simulink model "v0_pmsm_fsfb_sim_for_flipsky"  (R2025b)
settings: Solver=FixedStepAuto  StartTime=0.0  StopTime=inf  FixedStep=Ts_pwm  RelTol=1e-3
values from neighbouring files (symbols this model uses):
  Bv = pmsm.B    [mcb_pmsm_foc_qep_f28379d_SIUnit_data.m]    (also in mcb_pmsm_fsfb_f28379d_param.m = 2.636e-06; v0_pmsm_fsfb_sim_for_flipsky_.m = 9.444e-05; v1_0_3_sim_param_fsfc.m = 9.444e-05)
  C = [ 1, 0, 0 ... (first row only)    [mcb_pmsm_fsfb_f28379d_param.m]    (also in v0_pmsm_fsfb_sim_for_flipsky_.m = [; v1_0_3_sim_param_fsfc.m = [)
  J = 7.061e-6    (= 7.061e-06)    [mcb_pmsm_fsfb_f28379d_param.m]    (also in v0_pmsm_fsfb_sim_for_flipsky_.m = 0.00036179; v1_0_3_sim_param_fsfc.m = 0.00036179)
  Ki = -Ka_fsfb(2)    [mcb_pmsm_foc_qep_f28379d_SIUnit_data.m]    (also in mcb_pmsm_fsfb_f28379d_param.m = -K(:, n+1:end); v0_pmsm_fsfb_sim_for_flipsky_.m = -K(:, n+1:end); v1_0_3_sim_param_fsfc.m = -K(:, n+1:end))
  Kx = K(:, 1:n)    [mcb_pmsm_fsfb_f28379d_param.m]    (also in v0_pmsm_fsfb_sim_for_flipsky_.m; v1_0_3_sim_param_fsfc.m)
  L = Ld    (= 0.0002)    [mcb_pmsm_fsfb_f28379d_param.m]    (also in v0_pmsm_fsfb_sim_for_flipsky_.m = 0.0004; v1_0_3_sim_param_fsfc.m = 0.0013)
  Lambda_m = 0.01273    [mcb_pmsm_fsfb_f28379d_param.m]    (also in v0_pmsm_fsfb_sim_for_flipsky_.m = 0.0426; v1_0_3_sim_param_fsfc.m = 0.08627)
  P = 8    [mcb_pmsm_fsfb_f28379d_param.m]    (also in v0_pmsm_fsfb_sim_for_flipsky_.m; v1_0_3_sim_param_fsfc.m)
  Pk0 = 5e-4*diag([1e-3, 1e-2, 0.2, 0.01])    [v0_pmsm_fsfb_sim_for_flipsky_.m]    (also in v1_0_3_sim_param_fsfc.m)
  Qd = 1e-4*diag([0.5, 0.5, 5, 0.5])    [v0_pmsm_fsfb_sim_for_flipsky_.m]    (also in v1_0_3_sim_param_fsfc.m)
  R = Rs    (= 0.72)    [v0_pmsm_fsfb_sim_for_flipsky_.m]    (also in v1_0_3_sim_param_fsfc.m = 0.52)
  Rc = 56.33    [v0_pmsm_fsfb_sim_for_flipsky_.m]    (also in v1_0_3_sim_param_fsfc.m = 450)
  Rs = 0.3819    [mcb_pmsm_fsfb_f28379d_param.m]    (also in v0_pmsm_fsfb_sim_for_flipsky_.m = 0.72; v1_0_3_sim_param_fsfc.m = 0.52)
  Tc = 0.001    [v0_pmsm_fsfb_sim_for_flipsky_.m]    (also in v1_0_3_sim_param_fsfc.m)
  Ts = T_pwm    (= 5e-05)    [mcb_pmsm_foc_qep_f28379d_SIUnit_data.m]    (also in v0_pmsm_fsfb_sim_for_flipsky_.m = 0.0001; v1_0_3_sim_param_fsfc.m = 0.0001)
  X04 = 1e-2*[1; 1; 1; 0]    [v0_pmsm_fsfb_sim_for_flipsky_.m]    (also in v1_0_3_sim_param_fsfc.m)
libraries: simulink x4
settings Model: Creator=rotanakchhean  LastModifiedBy=LabPC

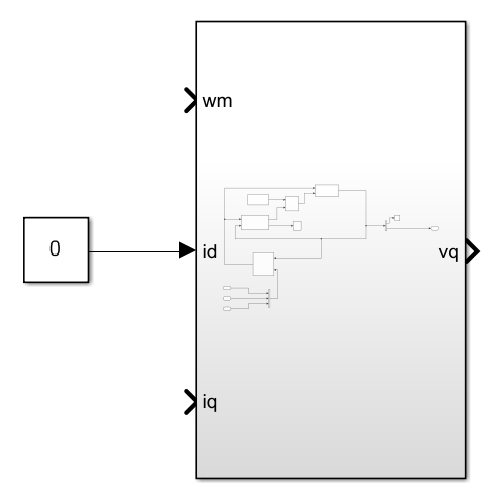
[thumbnail: Simulink's stored preview of the top-level diagram]
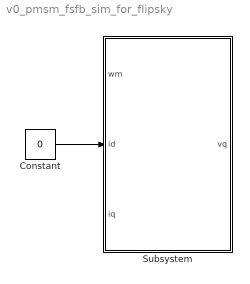
== system v0_pmsm_fsfb_sim_for_flipsky ==
  Constant : Constant  Value=0
  Subsystem : Subsystem
  wires:
  Constant/1 -> Subsystem/2(id)

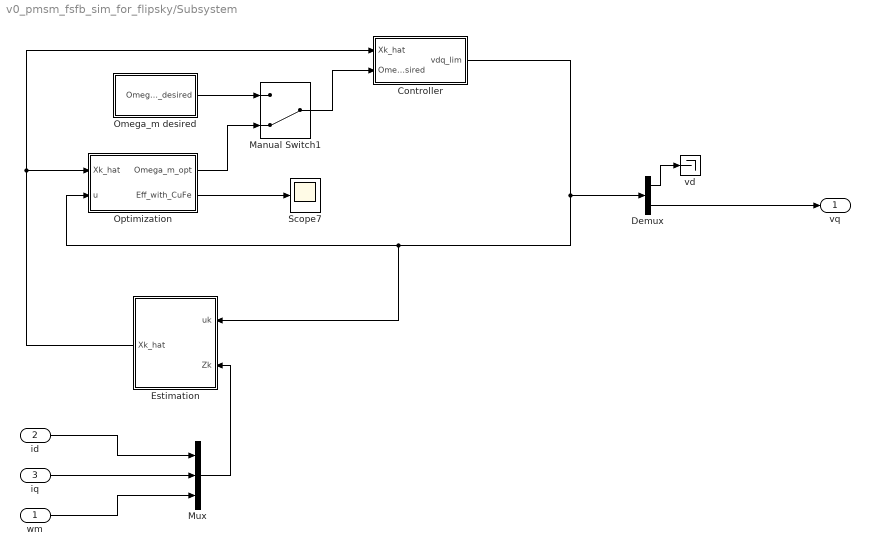
== system v0_pmsm_fsfb_sim_for_flipsky/Subsystem ==
  wm : Inport
  id : Inport  Port=2
  iq : Inport  Port=3
  Controller : Subsystem
  Demux : Demux  Outputs=2
  Estimation : Subsystem
  Manual Switch1 : ManualSwitch  CurrentSetting=0
  Mux : Mux  Inputs=3
  Omega_m desired : Subsystem
  Optimization : Subsystem
  Scope7 : Scope
      settings: ActiveDisplayYMinimum=-1.01629  ActiveDisplayYMaximum=1.19485
  vd : Terminator
  vq : Outport
  wires:
  Demux/2 -> vq/1
  wm/1 -> Mux/3
  Demux/1 -> vd/1
  Manual Switch1/1 -> Controller/2(Omega_m_desired)
  id/1 -> Mux/1
  Controller/1(vdq_lim) -> Demux/1, Optimization/2(u), Estimation/1(uk)
  Optimization/2(Eff_with_CuFe) -> Scope7/1
  Estimation/1(Xk_hat) -> Optimization/1(Xk_hat), Controller/1(Xk_hat)
  Optimization/1(Omega_m_opt) -> Manual Switch1/2
  Omega_m desired/1(Omega_m_desired) -> Manual Switch1/1
  iq/1 -> Mux/2
  Mux/1 -> Estimation/2(Zk)

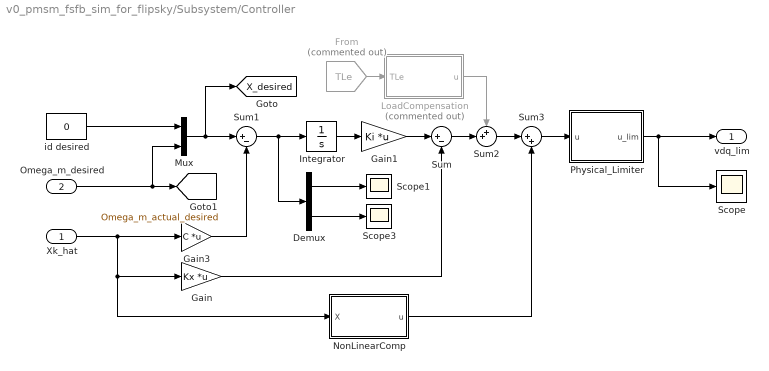
== system v0_pmsm_fsfb_sim_for_flipsky/Subsystem/Controller ==
  Xk_hat : Inport
  Omega_m_desired : Inport  Port=2
  Demux : Demux  Outputs=2
  From : From  Commented=on  GotoTag=TLe  TagVisibility=global
  Gain : Gain  Gain=Kx  Multiplication=Matrix(K*u)
  Gain1 : Gain  Gain=Ki  Multiplication=Matrix(K*u)
  Gain3 : Gain  Gain=C  Multiplication=Matrix(K*u)
  Integrator : Integrator
  LoadCompensation : MATLAB Function  Commented=on  TreatAsAtomicUnit=on
  Mux : Mux  Inputs=2
  NonLinearComp : MATLAB Function  TreatAsAtomicUnit=on
  Physical_Limiter : MATLAB Function  TreatAsAtomicUnit=on
  Scope : Scope
      settings: ActiveDisplayYMinimum=-1.5948  ActiveDisplayYMaximum=9.75273
  Scope1 : Scope
      settings: ActiveDisplayYMinimum=-0.02389  ActiveDisplayYMaximum=0.02118  DataLoggingVariableName=ScopeData2
  Scope3 : Scope
      settings: ActiveDisplayYMinimum=-0.06481  ActiveDisplayYMaximum=0.07204  DataLoggingVariableName=ScopeData4
  Sum : Sum  Inputs=|+-
  Sum1 : Sum  Inputs=|+-
  Sum2 : Sum  Inputs=++|
  Sum3 : Sum  Inputs=|++
  id desired : Constant  Value=0
  vdq_lim : Outport
  tag scope: Omega_m_actual_desired=global, X_desired=global
  wires:
  Gain1/1 -> Sum/1
  NonLinearComp/1(u) -> Sum3/2
  Gain/1 -> Sum/2
  Sum1/1 -> Integrator/1, Demux/1
  Sum/1 -> Sum2/2
  Integrator/1 -> Gain1/1
  Gain3/1 -> Sum1/2
  Omega_m_desired/1 -> Mux/2, [Omega_m_actual_desired]
  id desired/1 -> Mux/1
  Physical_Limiter/1(u_lim) -> Scope/1, vdq_lim/1
  Sum3/1 -> Physical_Limiter/1(u)
  LoadCompensation/1(u) -> Sum2/1
  Xk_hat/1 -> Gain/1, NonLinearComp/1(X), Gain3/1
  Sum2/1 -> Sum3/1
  Demux/1 -> Scope1/1
  From/1 -> LoadCompensation/1(TLe)
  Demux/2 -> Scope3/1
  Mux/1 -> [X_desired], Sum1/1

== system v0_pmsm_fsfb_sim_for_flipsky/Subsystem/Estimation ==
  uk : Inport
  Zk : Inport  Port=2
  EKF Estimation : Subsystem
  Xk_hat : Outport
  wires:
  EKF Estimation/1(Xk_hat) -> Xk_hat/1
  Zk/1 -> EKF Estimation/2(Zk)
  uk/1 -> EKF Estimation/1(uk)

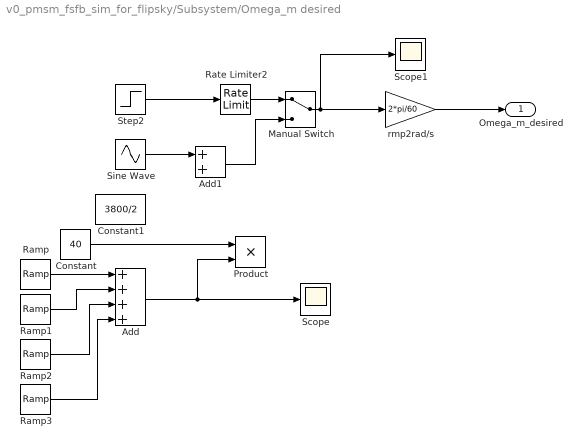
== system v0_pmsm_fsfb_sim_for_flipsky/Subsystem/Omega_m desired ==
  Add : Sum  Inputs=++++
  Add1 : Sum
  Constant : Constant  Value=40
  Constant1 : Constant  Value=3800/2
  Manual Switch : ManualSwitch
  Product : Product
  Ramp : simulink/Sources/Ramp  slope=1  start=5  InitialOutput=0
  Ramp1 : simulink/Sources/Ramp  slope=-1  start=15  InitialOutput=0
  Ramp2 : simulink/Sources/Ramp  slope=-1  start=35  InitialOutput=0
  Ramp3 : simulink/Sources/Ramp  slope=1  start=45  InitialOutput=0
  Rate Limiter2 : RateLimiter  RisingSlewLimit=700  FallingSlewLimit=-700  SampleTimeMode=inherited
  Scope : Scope
      settings: ActiveDisplayYMinimum=-1.25  ActiveDisplayYMaximum=11.25
  Scope1 : Scope
      settings: ActiveDisplayYMinimum=-23.34156  ActiveDisplayYMaximum=210.07406
  Sine Wave : Sin  Amplitude=3800  Frequency=2*pi*0.25  SampleTime=0
  Step2 : Step  Time=0  After=2200  SampleTime=0
  rmp2rad/s : Gain  Gain=2*pi/60
  Omega_m_desired : Outport
  wires:
  Rate Limiter2/1 -> Manual Switch/1
  rmp2rad/s/1 -> Omega_m_desired/1
  Sine Wave/1 -> Add1/1
  Step2/1 -> Rate Limiter2/1
  Ramp/1 -> Add/1
  Ramp1/1 -> Add/2
  Ramp2/1 -> Add/3
  Add/1 -> Product/2, Scope/1
  Ramp3/1 -> Add/4
  Constant/1 -> Product/1
  Manual Switch/1 -> Scope1/1, rmp2rad/s/1
  Add1/1 -> Manual Switch/2

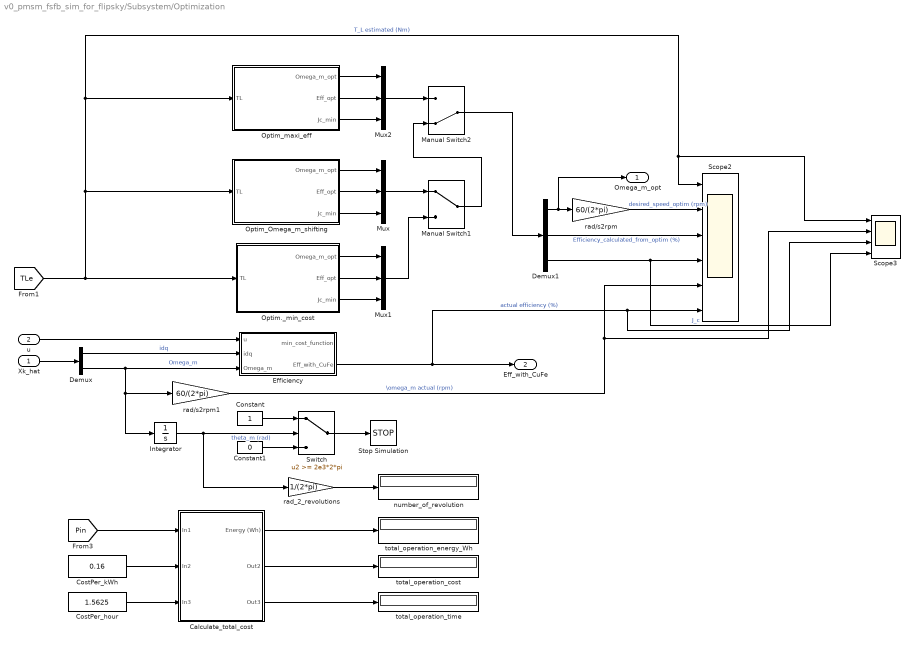
== system v0_pmsm_fsfb_sim_for_flipsky/Subsystem/Optimization ==
  Xk_hat : Inport
  u : Inport  Port=2
  Calculate_total_cost : Subsystem
  Constant : Constant
  Constant1 : Constant  Value=0
  CostPer_hour : Constant  Value=1.5625
  CostPer_kWh : Constant  Value=0.16
  Demux : Demux  Outputs=[2, 1]
  Demux1 : Demux  Outputs=3
  Efficiency : Subsystem
  Integrator : Integrator
  Manual Switch1 : ManualSwitch
  Manual Switch2 : ManualSwitch  CurrentSetting=0
  Mux : Mux  Inputs=3
  Mux1 : Mux  Inputs=3
  Mux2 : Mux  Inputs=3
  Optim._min_cost : MATLAB Function  TreatAsAtomicUnit=on
  Optim_Omega_m_shifting : MATLAB Function  TreatAsAtomicUnit=on
  Optim_maxi_eff : MATLAB Function  TreatAsAtomicUnit=on
  Scope2 : Scope  NumInputPorts=6
      settings: ActiveDisplayYMinimum=-0.6392  ActiveDisplayYMaximum=5.74724
  Scope3 : Scope  NumInputPorts=4
      settings: ActiveDisplayYMinimum=-0.64888  ActiveDisplayYMaximum=5.83743  YLabel=Torque (Nm)
  Stop Simulation : Stop
  Switch : Switch  Threshold=2e3*2*pi  SaturateOnIntegerOverflow=off  InputSameDT=off
  number_of_revolution : Display
  rad/s2rpm : Gain  Gain=60/(2*pi)
  rad/s2rpm1 : Gain  Gain=60/(2*pi)
  rad_2_revolutions : Gain  Gain=1/(2*pi)
  total_operation_cost : Display
  total_operation_energy_Wh : Display
  total_operation_time : Display
  Omega_m_opt : Outport
  Eff_with_CuFe : Outport  Port=2
  wires:
  Xk_hat/1 -> Demux/1
  u/1 -> Efficiency/1(u)
  Demux/1 -> Efficiency/2(idq)  "idq"
  Demux/2 -> Efficiency/3(Omega_m), Integrator/1, rad/s2rpm1/1  "Omega_m"
  rad/s2rpm/1 -> Scope2/2  "desired_speed_optim (rpm)"
  Efficiency/2(Eff_with_CuFe) -> Scope3/3, Scope2/6, Eff_with_CuFe/1  "actual efficiency (%)"
  Demux1/1 -> rad/s2rpm/1, Omega_m_opt/1
  [TLe] -> Optim._min_cost/1(TL), Optim_Omega_m_shifting/1(TL), Scope2/1, Scope3/1, Optim_maxi_eff/1(TL)  "T_L estimated (Nm)"
  rad/s2rpm1/1 -> Scope2/5, Scope3/2  "\\omega_m actual (rpm)"
  Integrator/1 -> Switch/2, rad_2_revolutions/1  "theta_m (rad)"
  Constant1/1 -> Switch/3
  Constant/1 -> Switch/1
  Calculate_total_cost/2(Out2) -> total_operation_cost/1
  [Pin] -> Calculate_total_cost/1(In1)
  CostPer_kWh/1 -> Calculate_total_cost/2(In2)
  CostPer_hour/1 -> Calculate_total_cost/3(In3)
  Calculate_total_cost/1(Energy (Wh)) -> total_operation_energy_Wh/1
  Calculate_total_cost/3(Out3) -> total_operation_time/1
  Optim_Omega_m_shifting/3(Jc_min) -> Mux/3
  Optim_Omega_m_shifting/2(Eff_opt) -> Mux/2
  Optim._min_cost/2(Eff_opt) -> Mux1/2
  Optim._min_cost/1(Omega_m_opt) -> Mux1/1
  Optim._min_cost/3(Jc_min) -> Mux1/3
  Mux/1 -> Manual Switch1/1
  Mux1/1 -> Manual Switch1/2
  Optim_Omega_m_shifting/1(Omega_m_opt) -> Mux/1
  Demux1/3 -> Scope3/4, Scope2/4  "J_c"
  rad_2_revolutions/1 -> number_of_revolution/1
  Optim_maxi_eff/1(Omega_m_opt) -> Mux2/1
  Optim_maxi_eff/2(Eff_opt) -> Mux2/2
  Optim_maxi_eff/3(Jc_min) -> Mux2/3
  Mux2/1 -> Manual Switch2/1
  Manual Switch1/1 -> Manual Switch2/2
  Manual Switch2/1 -> Demux1/1
  Demux1/2 -> Scope2/3  "Efficiency_calculated_from_optim (%)"
  Switch/1 -> Stop Simulation/1

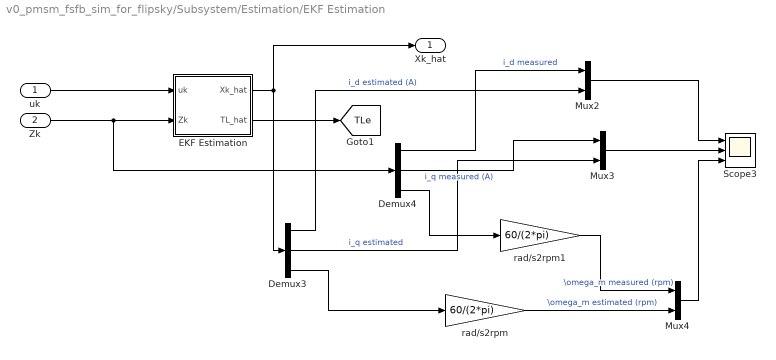
== system v0_pmsm_fsfb_sim_for_flipsky/Subsystem/Estimation/EKF Estimation ==
  uk : Inport
  Zk : Inport  Port=2
  Demux3 : Demux  Outputs=3
  Demux4 : Demux  Outputs=3
  EKF Estimation : Subsystem
  Mux2 : Mux  Inputs=2
  Mux3 : Mux  Inputs=2
  Mux4 : Mux  Inputs=2
  Scope3 : Scope  NumInputPorts=3
      settings: ActiveDisplayYMinimum=-2.79333  ActiveDisplayYMaximum=3.10469  YLabel=Current (A)  DataLoggingVariableName=ScopeData2
  rad/s2rpm : Gain  Gain=60/(2*pi)
  rad/s2rpm1 : Gain  Gain=60/(2*pi)
  Xk_hat : Outport
  tag scope: TLe=global
  wires:
  uk/1 -> EKF Estimation/1(uk)
  Demux3/3 -> rad/s2rpm/1
  EKF Estimation/1(Xk_hat) -> Xk_hat/1, Demux3/1
  Demux4/2 -> Mux3/1  "i_q measured (A)"
  Mux3/1 -> Scope3/2
  Demux3/1 -> Mux2/2  "i_d estimated (A)"
  Zk/1 -> Demux4/1, EKF Estimation/2(Zk)
  Demux4/3 -> rad/s2rpm1/1
  Mux2/1 -> Scope3/1
  Demux3/2 -> Mux3/2  "i_q estimated"
  EKF Estimation/2(TL_hat) -> [TLe]
  Demux4/1 -> Mux2/1  "i_d measured"
  Mux4/1 -> Scope3/3
  rad/s2rpm/1 -> Mux4/2  "\\omega_m estimated (rpm)"
  rad/s2rpm1/1 -> Mux4/1  "\\omega_m measured (rpm)"

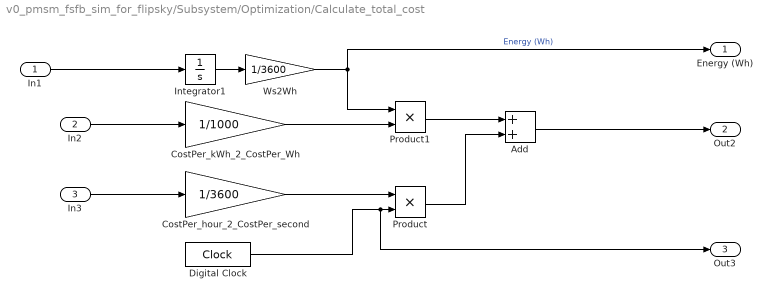
== system v0_pmsm_fsfb_sim_for_flipsky/Subsystem/Optimization/Calculate_total_cost ==
  In1 : Inport
  In2 : Inport  Port=2
  In3 : Inport  Port=3
  Add : Sum
  CostPer_hour_2_CostPer_second : Gain  Gain=1/3600
  CostPer_kWh_2_CostPer_Wh : Gain  Gain=1/1000
  Digital Clock : DigitalClock
  Integrator1 : Integrator
  Product : Product
  Product1 : Product
  Ws2Wh : Gain  Gain=1/3600
  Energy (Wh) : Outport
  Out2 : Outport  Port=2
  Out3 : Outport  Port=3
  wires:
  In1/1 -> Integrator1/1
  Add/1 -> Out2/1
  In3/1 -> CostPer_hour_2_CostPer_second/1
  CostPer_kWh_2_CostPer_Wh/1 -> Product1/2
  In2/1 -> CostPer_kWh_2_CostPer_Wh/1
  CostPer_hour_2_CostPer_second/1 -> Product/1
  Integrator1/1 -> Ws2Wh/1
  Product/1 -> Add/2
  Product1/1 -> Add/1
  Ws2Wh/1 -> Energy (Wh)/1, Product1/1  "Energy (Wh)"
  Digital Clock/1 -> Out3/1, Product/2

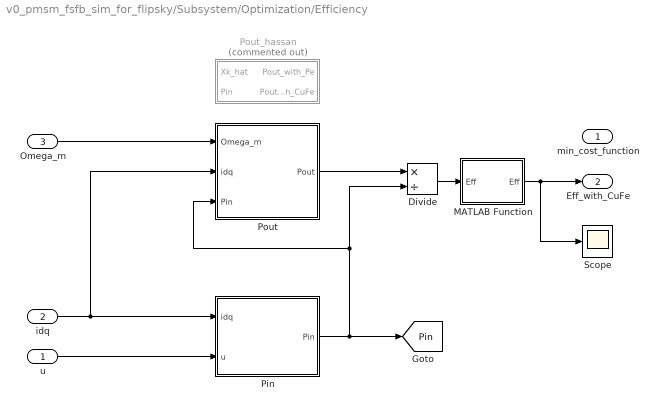
== system v0_pmsm_fsfb_sim_for_flipsky/Subsystem/Optimization/Efficiency ==
  u : Inport
  idq : Inport  Port=2
  Omega_m : Inport  Port=3
  Divide : Product  Inputs=*/
  MATLAB Function : MATLAB Function  TreatAsAtomicUnit=on
  Pin : Subsystem
  Pout : Subsystem
  Pout_hassan : Subsystem  Commented=on
  Scope : Scope
      settings: ActiveDisplayYMinimum=0.66193  ActiveDisplayYMaximum=1.02331  DataLoggingVariableName=ScopeData2
  min_cost_function : Outport
  Eff_with_CuFe : Outport  Port=2
  tag scope: Pin=global
  wires:
  idq/1 -> Pout/2(idq), Pin/1(idq)
  u/1 -> Pin/2(u)
  Pin/1(Pin) -> [Pin], Divide/2, Pout/3(Pin)
  Pout/1(Pout) -> Divide/1
  Divide/1 -> MATLAB Function/1("Eff ")
  Omega_m/1 -> Pout/1(Omega_m)
  MATLAB Function/1(Eff) -> Scope/1, Eff_with_CuFe/1

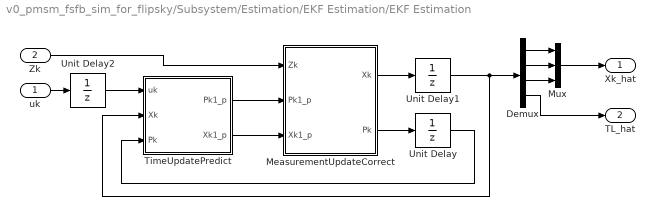
== system v0_pmsm_fsfb_sim_for_flipsky/Subsystem/Estimation/EKF Estimation/EKF Estimation ==
  uk : Inport
  Zk : Inport  Port=2
  Demux : Demux
  MeasurementUpdateCorrect : MATLAB Function  TreatAsAtomicUnit=on
  Mux : Mux  Inputs=3
  TimeUpdatePredict : MATLAB Function  TreatAsAtomicUnit=on
  Unit Delay : UnitDelay  InitialCondition=Pk0  SampleTime=-1  HasFrameUpgradeWarning=on
  Unit Delay1 : UnitDelay  InitialCondition=X04  SampleTime=-1  HasFrameUpgradeWarning=on
  Unit Delay2 : UnitDelay  SampleTime=-1  HasFrameUpgradeWarning=on
  Xk_hat : Outport
  TL_hat : Outport  Port=2
  wires:
  uk/1 -> Unit Delay2/1
  TimeUpdatePredict/1(Pk1_p) -> MeasurementUpdateCorrect/2(Pk1_p)
  TimeUpdatePredict/2(Xk1_p) -> MeasurementUpdateCorrect/3(Xk1_p)
  Zk/1 -> MeasurementUpdateCorrect/1(Zk)
  MeasurementUpdateCorrect/2(Pk) -> Unit Delay/1
  Unit Delay/1 -> TimeUpdatePredict/3(Pk)
  MeasurementUpdateCorrect/1(Xk) -> Unit Delay1/1
  Unit Delay1/1 -> Demux/1, TimeUpdatePredict/2(Xk)
  Demux/3 -> Mux/3
  Demux/2 -> Mux/2
  Demux/1 -> Mux/1
  Mux/1 -> Xk_hat/1
  Demux/4 -> TL_hat/1
  Unit Delay2/1 -> TimeUpdatePredict/1(uk)

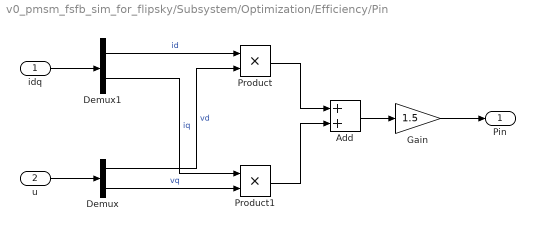
== system v0_pmsm_fsfb_sim_for_flipsky/Subsystem/Optimization/Efficiency/Pin ==
  idq : Inport
  u : Inport  Port=2
  Add : Sum
  Demux : Demux  Outputs=2
  Demux1 : Demux  Outputs=2
  Gain : Gain  Gain=1.5
  Product : Product
  Product1 : Product
  Pin : Outport
  wires:
  Product/1 -> Add/1
  Product1/1 -> Add/2
  Add/1 -> Gain/1
  Gain/1 -> Pin/1
  Demux1/1 -> Product/1  "id"
  Demux1/2 -> Product1/1  "iq"
  Demux/1 -> Product/2  "vd"
  Demux/2 -> Product1/2  "vq"
  u/1 -> Demux/1
  idq/1 -> Demux1/1

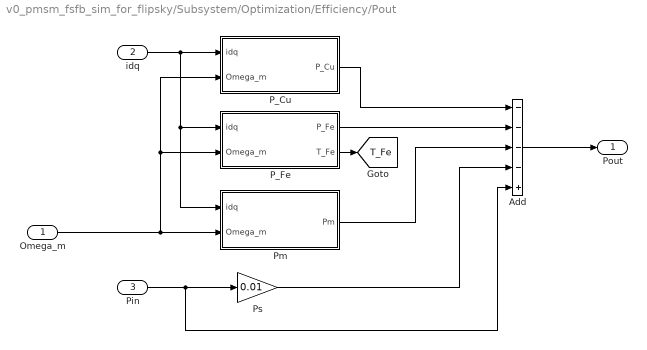
== system v0_pmsm_fsfb_sim_for_flipsky/Subsystem/Optimization/Efficiency/Pout ==
  Omega_m : Inport
  idq : Inport  Port=2
  Pin : Inport  Port=3
  Add : Sum  Inputs=----+
  P_Cu : MATLAB Function  TreatAsAtomicUnit=on
  P_Fe : MATLAB Function  TreatAsAtomicUnit=on
  Pm : MATLAB Function  TreatAsAtomicUnit=on
  Ps : Gain  Gain=0.01
  Pout : Outport
  tag scope: T_Fe=global
  wires:
  idq/1 -> Pm/1(idq), P_Fe/1(idq), P_Cu/1(idq)
  Pin/1 -> Ps/1, Add/5
  Ps/1 -> Add/4
  Pm/1(Pm) -> Add/3
  P_Fe/1(P_Fe) -> Add/2
  P_Cu/1(P_Cu) -> Add/1
  Add/1 -> Pout/1
  Omega_m/1 -> Pm/2(Omega_m), P_Cu/2(Omega_m), P_Fe/2(Omega_m)
  P_Fe/2(T_Fe) -> [T_Fe]

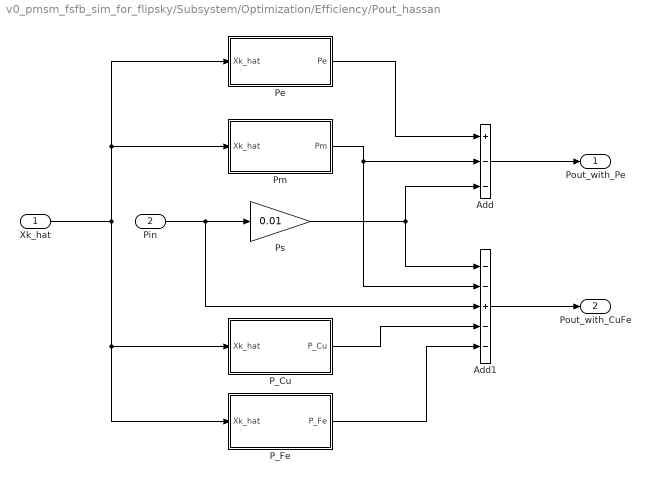
== system v0_pmsm_fsfb_sim_for_flipsky/Subsystem/Optimization/Efficiency/Pout_hassan ==
  Xk_hat : Inport
  Pin : Inport  Port=2
  Add : Sum  Inputs=+--
  Add1 : Sum  Inputs=--+--
  P_Cu : MATLAB Function  TreatAsAtomicUnit=on
  P_Fe : MATLAB Function  TreatAsAtomicUnit=on
  Pe : MATLAB Function  TreatAsAtomicUnit=on
  Pm : MATLAB Function  TreatAsAtomicUnit=on
  Ps : Gain  Gain=0.01
  Pout_with_Pe : Outport
  Pout_with_CuFe : Outport  Port=2
  wires:
  Pin/1 -> Add1/3, Ps/1
  Pe/1(Pe) -> Add/1
  Pm/1(Pm) -> Add/2, Add1/2
  Ps/1 -> Add1/1, Add/3
  Add/1 -> Pout_with_Pe/1
  Xk_hat/1 -> Pe/1(Xk_hat), Pm/1(Xk_hat), P_Fe/1(Xk_hat), P_Cu/1(Xk_hat)
  P_Cu/1(P_Cu) -> Add1/4
  P_Fe/1(P_Fe) -> Add1/5
  Add1/1 -> Pout_with_CuFe/1

== matlab function v0_pmsm_fsfb_sim_for_flipsky/Subsystem/Controller/LoadCompensation ==
  data: TLe input; u output; P parameter; R parameter; Lambda_m parameter
function u = fcn(TLe, P, R, Lambda_m)

u = [
        0;
        4*R/(3*P*Lambda_m)*TLe;
    ];

== matlab function v0_pmsm_fsfb_sim_for_flipsky/Subsystem/Controller/NonLinearComp ==
  data: X input size=[3 1]; u output; P parameter; L parameter
function u = fcn(X, P, L)

id = X(1);
iq = X(2);
wm = X(3);

u = [
        -P/2*L*wm*iq;
        P/2*L*wm*id;
    ];

== matlab function v0_pmsm_fsfb_sim_for_flipsky/Subsystem/Optimization/Efficiency/Pout/P_Cu ==
  data: idq input; P_Cu output; Rc parameter; Lambda_m parameter; L parameter; P parameter; Rs parameter; Omega_m input
function P_Cu = fcn(idq, Rc, Lambda_m, L, P, Rs, Omega_m)

id = idq(1);
iq = idq(2);
Omega_e = Omega_m*P/2;

Iod_num = Rc^2*id + Rc*L*Omega_e*iq - L*Omega_e^2*Lambda_m;
Iod_denum = Rc^2 + (L*Omega_e)^2;
Iod = Iod_num/Iod_denum;

Ioq_num = Rc*(Rc*iq - Lambda_m*Omega_e - L*id*Omega_e);
Ioq_denum = Iod_denum;
Ioq = Ioq_num/Ioq_denum;

factor = (3/2)*Rs;
term1 = Iod - (Omega_e*L*Ioq/Rc);
term2 = Ioq + Omega_e*(Lambda_m + L*Iod)/Rc;

P_Cu = factor*(term1^2 + term2^2);

== matlab function v0_pmsm_fsfb_sim_for_flipsky/Subsystem/Optimization/Efficiency/Pout/P_Fe ==
  data: idq input; P_Fe output; Rc parameter; Lambda_m parameter; L parameter; P parameter; Omega_m input; T_Fe output
function [P_Fe, T_Fe] = fcn(idq, Rc, Lambda_m, L, P, Omega_m)

id = idq(1);
iq = idq(2);
Omega_e = Omega_m*P/2;

Iod_num = Rc^2*id + Rc*L*Omega_e*iq - L*Omega_e^2*Lambda_m;
Iod_denum = Rc^2 + (L*Omega_e)^2;
Iod = Iod_num/Iod_denum;

Ioq_num = Rc*(Rc*iq - Lambda_m*Omega_e - L*id*Omega_e);
Ioq_denum = Iod_denum;
Ioq = Ioq_num/Ioq_denum;

factor = (3/2)*(Omega_e^2/Rc);
term1 = L*Ioq;
term2 = Lambda_m + L*Iod;

P_Fe = factor*(term1^2 + term2^2);

factor1 = (3/2)*(Omega_e/Rc);
T_Fe = factor1*(term1^2 + term2^2)*P/2;

== matlab function v0_pmsm_fsfb_sim_for_flipsky/Subsystem/Optimization/Efficiency/Pout/Pm ==
  data: idq input; P parameter; Pm output; Tc parameter; Bv parameter; Omega_m input
function Pm = fcn(idq,P, Tc, Bv, Omega_m)

id = idq(1);
iq = idq(2);
Omega_e = Omega_m*P/2;


term1 = 4*Bv*Omega_e^2/P^2;
term2 = 2*Tc*Omega_e/P;

Pm = term1 + term2;

== matlab function v0_pmsm_fsfb_sim_for_flipsky/Subsystem/Optimization/Efficiency/Pout_hassan/P_Cu ==
  data: Xk_hat input; P_Cu output; Lambda_m parameter; L parameter; Rc parameter; P parameter; R parameter
function P_Cu = fcn(Xk_hat, Lambda_m, L, Rc, P, R)
id = Xk_hat(1);
iq = Xk_hat(2);
Omega_m = Xk_hat(3);
Omega_e = Omega_m*P/2;

factor = (3/2)*R;
denominator = (Rc^2 + (L*Omega_e)^2);

term1 = (Rc^2*id + Rc*L*Omega_e*iq - L*Omega_e^2*Lambda_m)/denominator;

term2 = Omega_e*L*(Rc*iq - Lambda_m*Omega_e - L*id*Omega_e)/denominator;

term3 = Rc*(Rc*iq - Lambda_m*Omega_e - L*id*Omega_e)/denominator;

term4 = (Omega_e/Rc)*(Lambda_m + L*term1);

P_Cu = factor * ((term1 - term2)^2 + (term3 + term4)^2);

== matlab function v0_pmsm_fsfb_sim_for_flipsky/Subsystem/Optimization/Efficiency/Pout_hassan/P_Fe ==
  data: Xk_hat input; P_Fe output; Lambda_m parameter; L parameter; Rc parameter; P parameter
function P_Fe = fcn(Xk_hat, Lambda_m, L, Rc, P)
id = Xk_hat(1);
iq = Xk_hat(2);
Omega_m = Xk_hat(3);
Omega_e = Omega_m*P/2;

factor = (3/2)*Omega_e^2/Rc;

term1 = L*Rc*(Rc*iq - Lambda_m*Omega_e - L*id*Omega_e)/(Rc^2 + (L*Omega_e)^2);
term2 = Lambda_m + L*(Rc^2*id + Rc*L*Omega_e*iq - L*Omega_e^2*Lambda_m)/(Rc^2 + (L*Omega_e)^2);

P_Fe = factor * (term1^2 + term2^2);

== matlab function v0_pmsm_fsfb_sim_for_flipsky/Subsystem/Optimization/Efficiency/Pout_hassan/Pe ==
  data: Xk_hat input; Pe output; Lambda_m parameter; L parameter; Rc parameter; P parameter
function Pe = fcn(Xk_hat, Lambda_m, L, Rc, P)
id = Xk_hat(1);
iq = Xk_hat(2);
Omega_m = Xk_hat(3);
Omega_e = Omega_m*P/2;
factor = 3*P*Lambda_m*Rc*Omega_e/4;
numerator = Rc*iq - Lambda_m*Omega_e - L*id*Omega_e;
denomiator = Rc^2 + (L*Omega_e)^2;

Pe = factor*numerator/denomiator;

== matlab function v0_pmsm_fsfb_sim_for_flipsky/Subsystem/Optimization/Efficiency/Pout_hassan/Pm ==
  data: Xk_hat input; Pm output; Bv parameter; Tc parameter; P parameter
function Pm = fcn(Xk_hat, Bv, Tc, P)
% id = Xk_hat(1);
% iq = Xk_hat(2);
Omega_m = Xk_hat(3);
Omega_e = Omega_m*P/2;

Pm = (4/P^2)*Bv*Omega_e^2 + (2/P)*Tc*Omega_e;

== matlab function v0_pmsm_fsfb_sim_for_flipsky/Subsystem/Controller/Physical_Limiter ==
  data: u input; u_lim output; Vdc parameter
function u_lim = fcn(u, Vdc)
    vd = u(1);
    vq = u(2);
    V_max = Vdc/sqrt(3);

    V_mag = sqrt(vd^2 + vq^2);

    if V_mag > V_max
        scale = V_max / V_mag;
        vd_lim = vd * scale;
        vq_lim = vq * scale;
    else
        vd_lim = vd;
        vq_lim = vq;
    end
    u_lim  = [vd_lim; vq_lim];

== matlab function v0_pmsm_fsfb_sim_for_flipsky/Subsystem/Optimization/Efficiency/MATLAB Function ==
  data: Eff input; Eff output
function Eff = fcn(Eff)

if Eff < 0.2
    Eff = 0.2;
elseif Eff > 1
    Eff = 1;
end
Eff = Eff*100;

== matlab function v0_pmsm_fsfb_sim_for_flipsky/Subsystem/Optimization/Optim_Omega_m_shifting ==
  data: Omega_m_opt output; Eff_opt output; Jc_min output; TL input; Rc parameter; Lambda_m parameter; L parameter; P parameter; Rs parameter; Tc parameter; Bv parameter; J parameter
function [Omega_m_opt, Eff_opt, Jc_min] = fcn(TL, Rc, Lambda_m, L, P, Rs, Tc, Bv, J)

Omega_m_min = 500; %rpm
Omega_m_max = 5000; %rmp

Omega_m_min = Omega_m_min*2*pi/60; %rad/s
Omega_m_max = Omega_m_max*2*pi/60; %rad/s

Omega_e_min = (P/2)*Omega_m_min*2*pi/60; %rad/s
Omega_e_max = (P/2)*Omega_m_max*2*pi/60; %rad/s

%% Method 1

% Eff_opt = 0;
% Omega_e_opt = Omega_m_max*P/2;
% for Omega_m = linspace(Omega_m_min, Omega_m_max, 1000)
%     Omega_e = Omega_m*P/2;
%      Eff_opt_calc = Calculate_Eff(Omega_e, idq, u, Rc, Lambda_m, L, P, Rs, Tc, Bv);
%      if Eff_opt_calc > Eff_opt
%          Eff_opt = Eff_opt_calc;
%          Omega_e_opt = Omega_e;
%      end
% end
%% Method 2
% Omega_m_a = Omega_m_min;
% Omega_e_a = Omega_m_a*P/2;
% 
% Omega_m_b = Omega_m_max;
% Omega_e_b = Omega_m_b*P/2;
% 
% a = Omega_e_a;
% b = Omega_e_b;
% tol = 1e-4;
% 
% for i = 1:500
%     c = (a+b)/2;
%     dEff_c = Calculate_dEff(c, idq, u, Rc, Lambda_m, L, P, Rs, Tc, Bv);
% 
%     if abs(b - a) < tol
%         break;
%     end
% 
%     if dEff_c > 0
%         a = c;
%     else
%         b = c;
%     end
% 
% end
% Compute optimal Omega_m_opt
% Omega_e_opt = (a + b) / 2;
%% Method 3
alpha = 0.75;
theta_e = 2*pi*100;
Eff_1min = 10;
Eff_1max = 100;

Omega_e = linspace(0, 0, 1000);
Eff = linspace(0, 0, 1000);
Jc = linspace(0, 0, 1000);
i = 0;
for Omega_m = linspace(Omega_m_min, Omega_m_max, 1000)
    i = i+1;
    Omega_e(i) = Omega_m*P/2;
    Eff(i) = Calculate_Eff(Omega_e(i), TL, Rc, Lambda_m, L, P, Rs, Tc, Bv, J);
    Eff_1n = (Eff(i) - Eff_1min)/(Eff_1max - Eff_1min);
    Eff_1n = 1/Eff_1n;
    t_min = theta_e/Omega_e_max;
    t_max = theta_e/Omega_e_min;
    t = theta_e/Omega_e(i);
    t_n = (t - t_min)/(t_max - t_min);
    Jc(i) = alpha*Eff_1n + (1 - alpha)*t_n;

end
[Jc_min, Jc_idx] = min(Jc);
Omega_e_opt = Omega_e(Jc_idx);
Omega_m_opt = Omega_e_opt * 2 / P;
Eff_opt = Eff(Jc_idx);


if Eff_opt < 0.2
    Eff_opt = 0.2;
elseif Eff_opt > 1
    Eff_opt = 1;
end
Eff_opt = Eff_opt*100;



%% Calculate Pin
function Eff = Calculate_Eff(Omega_e, TL, Rc, Lambda_m, L, P, Rs, Tc, Bv, J)
    
    % dt = 0.00001;
    % Omega_e_dot = (Omega_e - Omega_e_dot)/dt;
    Omega_e_dot = 0;
    id = 0;

    Te = J*Omega_e_dot*2/P + TL + Bv*Omega_e*2/P;
    % iq = Te*4/(3*P*Lambda_m);

    iq = 4*Te*(Rc^2 + (L*Omega_e)^2)/(3*P*Lambda_m*Rc^2) + (Lambda_m*Omega_e - L*id*Omega_e)/Rc;

    % Calculate P_e
    P_e = Te*Omega_e*2/P;
    
    % Calculate P_Fe
    Iod_num = Rc^2*id + Rc*L*Omega_e*iq - L*Omega_e^2*Lambda_m;
    Iod_denum = Rc^2 + (L*Omega_e)^2;
    Iod = Iod_num/Iod_denum;
    
    Ioq_num = Rc*(Rc*iq - Lambda_m*Omega_e - L*id*Omega_e);
    Ioq_denum = Iod_denum;
    Ioq = Ioq_num/Ioq_denum;
    
    factor = (3/2)*(Omega_e^2/Rc);
    term1 = L*Ioq;
    term2 = Lambda_m + L*Iod;
    
    P_Fe = factor*(term1^2 + term2^2);
    
    % Calculate P_Cu
    factor_cu = (3/2)*Rs;
    term1_cu = Iod - (Omega_e*L*Ioq/Rc);
    term2_cu = Ioq + Omega_e*(Lambda_m + L*Iod)/Rc;
    
    P_Cu = factor_cu*(term1_cu^2 + term2_cu^2);
    
    % Calculate P_s
    P_s = 0.01*(P_Cu + P_Fe + P_e);
    
    % Calculate P_m
    term1_m = 4*Bv*Omega_e^2/P^2;
    term2_m = 2*Tc*Omega_e/P;
    
    P_m = term1_m + term2_m;
    
    % Calculate P_in
    P_in = P_Cu + P_Fe + P_e;
    % Calculate Efficiency
    Eff = (P_e - P_m - P_s)/P_in;
    if Eff >= 1
        Eff = 1;
    elseif Eff <= 0.1
        Eff = 10;
    end
    Eff = 100*Eff;


% %% Calculate dEfficiency
% function dEff_dWe = Calculate_dEff(Omega_e, TL, Rc, Lambda_m, L, P, Rs, Tc, Bv, J, Omega_e_dot)
% 
%     Eff1 = Calculate_Eff(Omega_e, TL, Rc, Lambda_m, L, P, Rs, Tc, Bv, J, Omega_e_dot);
%     Eff2 = Calculate_Eff(Omega_e, TL, Rc, Lambda_m, L, P, Rs, Tc, Bv, J, Omega_e_dot);
%     dOmega_e = Omega_e - Omega_e_dot;
%     dEff_dWe = (Eff2 - Eff1)/dOmega_e;


%% Calculate Omega_e_dot

== matlab function v0_pmsm_fsfb_sim_for_flipsky/Subsystem/Optimization/Optim_maxi_eff ==
  data: Omega_m_opt output; Eff_opt output; Jc_min output; TL input; Rc parameter; Lambda_m parameter; L parameter; P parameter; Rs parameter; Tc parameter; Bv parameter; J parameter
function [Omega_m_opt, Eff_opt, Jc_min] = fcn(TL, Rc, Lambda_m, L, P, Rs, Tc, Bv, J)

Omega_m_min = 500; %rpm
Omega_m_max = 5000; %rmp

Omega_m_min = Omega_m_min*2*pi/60; %rad/s
Omega_m_max = Omega_m_max*2*pi/60; %rad/s

Omega_e_min = (P/2)*Omega_m_min*2*pi/60; %rad/s
Omega_e_max = (P/2)*Omega_m_max*2*pi/60; %rad/s

%% Method 1

% Eff_opt = 0;
% Omega_e_opt = Omega_m_max*P/2;
% for Omega_m = linspace(Omega_m_min, Omega_m_max, 1000)
%     Omega_e = Omega_m*P/2;
%      Eff_opt_calc = Calculate_Eff(Omega_e, idq, u, Rc, Lambda_m, L, P, Rs, Tc, Bv);
%      if Eff_opt_calc > Eff_opt
%          Eff_opt = Eff_opt_calc;
%          Omega_e_opt = Omega_e;
%      end
% end
%% Method 2
% Omega_m_a = Omega_m_min;
% Omega_e_a = Omega_m_a*P/2;
% 
% Omega_m_b = Omega_m_max;
% Omega_e_b = Omega_m_b*P/2;
% 
% a = Omega_e_a;
% b = Omega_e_b;
% tol = 1e-4;
% 
% for i = 1:500
%     c = (a+b)/2;
%     dEff_c = Calculate_dEff(c, idq, u, Rc, Lambda_m, L, P, Rs, Tc, Bv);
% 
%     if abs(b - a) < tol
%         break;
%     end
% 
%     if dEff_c > 0
%         a = c;
%     else
%         b = c;
%     end
% 
% end
% Compute optimal Omega_m_opt
% Omega_e_opt = (a + b) / 2;
%% Method 3
alpha = 1;
theta_e = 2*pi*100;
Eff_1min = 10;
Eff_1max = 100;

Omega_e = linspace(0, 0, 1000);
Eff = linspace(0, 0, 1000);
i = 0;
for Omega_m = linspace(Omega_m_min, Omega_m_max, 1000)
    i = i+1;
    Omega_e(i) = Omega_m*P/2;
    Eff(i) = Calculate_Eff(Omega_e(i), TL, Rc, Lambda_m, L, P, Rs, Tc, Bv, J);
end
[Eff_max, Eff_idx] = max(Eff);
Omega_e_opt = Omega_e(Eff_idx);
Omega_m_opt = Omega_e_opt * 2 / P;
Eff_opt = Eff_max;
Jc_min = 0;

if Eff_opt < 0.2
    Eff_opt = 0.2;
elseif Eff_opt > 1
    Eff_opt = 1;
end
Eff_opt = Eff_opt*100;



%% Calculate Pin
function Eff = Calculate_Eff(Omega_e, TL, Rc, Lambda_m, L, P, Rs, Tc, Bv, J)
    
    % dt = 0.00001;
    % Omega_e_dot = (Omega_e - Omega_e_dot)/dt;
    Omega_e_dot = 0;
    id = 0;

    Te = J*Omega_e_dot*2/P + TL + Bv*Omega_e*2/P;
    % iq = Te*4/(3*P*Lambda_m);

    iq = 4*Te*(Rc^2 + (L*Omega_e)^2)/(3*P*Lambda_m*Rc^2) + (Lambda_m*Omega_e - L*id*Omega_e)/Rc;

    % Calculate P_e
    P_e = Te*Omega_e*2/P;
    
    % Calculate P_Fe
    Iod_num = Rc^2*id + Rc*L*Omega_e*iq - L*Omega_e^2*Lambda_m;
    Iod_denum = Rc^2 + (L*Omega_e)^2;
    Iod = Iod_num/Iod_denum;
    
    Ioq_num = Rc*(Rc*iq - Lambda_m*Omega_e - L*id*Omega_e);
    Ioq_denum = Iod_denum;
    Ioq = Ioq_num/Ioq_denum;
    
    factor = (3/2)*(Omega_e^2/Rc);
    term1 = L*Ioq;
    term2 = Lambda_m + L*Iod;
    
    P_Fe = factor*(term1^2 + term2^2);
    
    % Calculate P_Cu
    factor_cu = (3/2)*Rs;
    term1_cu = Iod - (Omega_e*L*Ioq/Rc);
    term2_cu = Ioq + Omega_e*(Lambda_m + L*Iod)/Rc;
    
    P_Cu = factor_cu*(term1_cu^2 + term2_cu^2);
    
    % Calculate P_s
    P_s = 0.01*(P_Cu + P_Fe + P_e);
    
    % Calculate P_m
    term1_m = 4*Bv*Omega_e^2/P^2;
    term2_m = 2*Tc*Omega_e/P;
    
    P_m = term1_m + term2_m;
    
    % Calculate P_in
    P_in = P_Cu + P_Fe + P_e;
    % Calculate Efficiency
    Eff = (P_e - P_m - P_s)/P_in;
    % if Eff >= 1
    %     Eff = 1;
    % elseif Eff <= 0.1
    %     Eff = 10;
    % end
    % Eff = 100*Eff;


% %% Calculate dEfficiency
% function dEff_dWe = Calculate_dEff(Omega_e, TL, Rc, Lambda_m, L, P, Rs, Tc, Bv, J, Omega_e_dot)
% 
%     Eff1 = Calculate_Eff(Omega_e, TL, Rc, Lambda_m, L, P, Rs, Tc, Bv, J, Omega_e_dot);
%     Eff2 = Calculate_Eff(Omega_e, TL, Rc, Lambda_m, L, P, Rs, Tc, Bv, J, Omega_e_dot);
%     dOmega_e = Omega_e - Omega_e_dot;
%     dEff_dWe = (Eff2 - Eff1)/dOmega_e;


%% Calculate Omega_e_dot

== matlab function v0_pmsm_fsfb_sim_for_flipsky/Subsystem/Optimization/Optim._min_cost ==
  data: Omega_m_opt output; TL input; Eff_opt output; Rc parameter; Lambda_m parameter; L parameter; P parameter; Rs parameter; Tc parameter; Bv parameter; J parameter; Jc_min output
function [Omega_m_opt, Eff_opt, Jc_min] = fcn(TL, Rc, Lambda_m, L, P, Rs, Tc, Bv, J)

Omega_m_min = 500; %rpm
Omega_m_max = 5000; %rmp

Omega_m_min = Omega_m_min*2*pi/60; %rad/s
Omega_m_max = Omega_m_max*2*pi/60; %rad/s

Omega_e_min = (P/2)*Omega_m_min*2*pi/60; %rad/s
Omega_e_max = (P/2)*Omega_m_max*2*pi/60; %rad/s

%% Method 1
theta_e = 100*2*pi;
a_e = 0.16; % $/kWh (range 0.12$ to 0.16$)
a_t = 1.5625; % $/h -> Labor cost

Omega_e = linspace(0, 0, 1000);
Eff = linspace(0, 0, 1000);
Jc = linspace(0, 0, 1000);
i = 0;
for Omega_m = linspace(Omega_m_min, Omega_m_max, 1000)
    i = i+1;
    Omega_e(i) = Omega_m*P/2;
    [Eff(i), P_in] = Calculate_Eff(Omega_e(i), TL, Rc, Lambda_m, L, P, Rs, Tc, Bv, J);
    Ce = 27e-8*a_e;
    Ct = 27e-5*a_t;
    Jc(i) = P_in*theta_e/Omega_e(i)*Ce + theta_e/Omega_e(i)*Ct;
end
[Jc_min, Jc_idx] = min(Jc);
Omega_e_opt = Omega_e(Jc_idx);
Omega_m_opt = Omega_e_opt * 2 / P;
Eff_opt = Eff(Jc_idx);


if Eff_opt < 0.2
    Eff_opt = 0.2;
elseif Eff_opt > 1
    Eff_opt = 1;
end
Eff_opt = Eff_opt*100;




%% Calculate Pin
function [Eff, P_in] = Calculate_Eff(Omega_e, TL, Rc, Lambda_m, L, P, Rs, Tc, Bv, J)
    
    % dt = 0.00001;
    % Omega_e_dot = (Omega_e - Omega_e_dot)/dt;
    Omega_e_dot = 0;
    id = 0;

    Te = J*Omega_e_dot*2/P + TL + Bv*Omega_e*2/P;
    % iq = Te*4/(3*P*Lambda_m);

    iq = 4*Te*(Rc^2 + (L*Omega_e)^2)/(3*P*Lambda_m*Rc^2) + (Lambda_m*Omega_e - L*id*Omega_e)/Rc;

    % Calculate P_e
    P_e = Te*Omega_e*2/P;
    
    % Calculate P_Fe
    Iod_num = Rc^2*id + Rc*L*Omega_e*iq - L*Omega_e^2*Lambda_m;
    Iod_denum = Rc^2 + (L*Omega_e)^2;
    Iod = Iod_num/Iod_denum;
    
    Ioq_num = Rc*(Rc*iq - Lambda_m*Omega_e - L*id*Omega_e);
    Ioq_denum = Iod_denum;
    Ioq = Ioq_num/Ioq_denum;
    
    factor = (3/2)*(Omega_e^2/Rc);
    term1 = L*Ioq;
    term2 = Lambda_m + L*Iod;
    
    P_Fe = factor*(term1^2 + term2^2);
    
    % Calculate P_Cu
    factor_cu = (3/2)*Rs;
    term1_cu = Iod - (Omega_e*L*Ioq/Rc);
    term2_cu = Ioq + Omega_e*(Lambda_m + L*Iod)/Rc;
    
    P_Cu = factor_cu*(term1_cu^2 + term2_cu^2);
    
    % Calculate P_s
    P_s = 0.01*(P_Cu + P_Fe + P_e);
    
    % Calculate P_m
    term1_m = 4*Bv*Omega_e^2/P^2;
    term2_m = 2*Tc*Omega_e/P;
    
    P_m = term1_m + term2_m;
    
    % Calculate P_in
    P_in = P_Cu + P_Fe + P_e;
    % Calculate Efficiency
    Eff = (P_e - P_m - P_s)/(P_Cu + P_Fe + P_e);
    if Eff >= 1
        Eff = 1;
    elseif Eff <= 0.1
        Eff = 10;
    end
    Eff = 100*Eff;


% %% Calculate dEfficiency
% function dEff_dWe = Calculate_dEff(Omega_e, TL, Rc, Lambda_m, L, P, Rs, Tc, Bv, J, Omega_e_dot)
% 
%     Eff1 = Calculate_Eff(Omega_e, TL, Rc, Lambda_m, L, P, Rs, Tc, Bv, J, Omega_e_dot);
%     Eff2 = Calculate_Eff(Omega_e, TL, Rc, Lambda_m, L, P, Rs, Tc, Bv, J, Omega_e_dot);
%     dOmega_e = Omega_e - Omega_e_dot;
%     dEff_dWe = (Eff2 - Eff1)/dOmega_e;


%% Calculate Omega_e_dot

== matlab function v0_pmsm_fsfb_sim_for_flipsky/Subsystem/Estimation/EKF Estimation/EKF Estimation/MeasurementUpdateCorrect ==
  data: Zk input; Pk1_p input; Xk1_p input; Xk output; Pk output; Rd parameter
function [Xk, Pk] = fcn(Zk, Pk1_p, Xk1_p, Rd)

Hjk = [
        1, 0, 0, 0;
        0, 1, 0, 0;
        0, 0, 1, 0;
    ];


Kk = Pk1_p*Hjk'/(Hjk*Pk1_p*Hjk' + Rd);

Xk = Xk1_p + Kk*(Zk - Hjk*Xk1_p);

Pk = (eye(4) - Kk*Hjk)*Pk1_p;

== matlab function v0_pmsm_fsfb_sim_for_flipsky/Subsystem/Estimation/EKF Estimation/EKF Estimation/TimeUpdatePredict ==
  data: Pk1_p output; uk input; Xk1_p output; Xk input size=[4 1]; Pk input size=[4 4]; Qd parameter; Bv parameter; J parameter; Lambda_m parameter; P parameter; L parameter; R parameter; Ts parameter
function [Pk1_p, Xk1_p] = fcn(uk, Xk, Pk, Qd, Bv, J, Lambda_m, P, L, R, Ts)
id = Xk(1);
iq = Xk(2);
wm = Xk(3);

%Predict the state ahead
Ad = [
        -R/L, P/2*wm, 0, 0;
        -P/2*wm, -R/L, -P/2*Lambda_m/L, 0;
        0, 3*P/4*Lambda_m/J, -Bv/J, -1/J;
        0, 0, 0, 0;
    ];
Bd = [
        1/L, 0;
        0, 1/L;
        0, 0;
        0, 0;
    ];
Adk = eye(4) + Ts*Ad;
Bdk = Ts*Bd;

Xk1_p = Adk*Xk + Bdk*uk;

%Predict the error covariance ahead
Aj = [
        -R/L, P/2*wm, P/2*iq, 0;
        -P/2*wm, -R/L, -P/2*(Lambda_m/L+id), 0;
        0, 3*P/4*Lambda_m/J, -Bv/J, -1/J;
        0, 0, 0, 0;
    ];

Ajk = eye(4) + Ts*Aj;

Pk1_p = Ajk*Pk*Ajk' + Ts*Qd;
